simulink model "Steppermotor"  (R2025b)
settings: Solver=FixedStepAuto  StartTime=0.0  StopTime=inf  FixedStep=0.05  RelTol=1e-3  EnableMultiTasking=on
libraries: raspberrypiBasiclib x5, simulink x3, raspberrypiNetworklib x1
settings Model: ExtModeTrigDuration=2  Creator=ioannisgeorgilas  LastModifiedBy=maiaguo
settings SolverCC: PositivePriorityOrder=on
settings OptimizationCC: EnhancedBackFolding=on  PassReuseOutputArgsAs=Individual arguments  ZeroExternalMemoryAtStartup=off  ZeroInternalMemoryAtStartup=off  MaxStackSize=200000  OptimizeBlockOrder=speed  DifferentSizesBufferReuse=on  OptimizationCustomize=off  EfficientTunableParamExpr=on
settings DebuggingCC: ParameterTunabilityLossMsg=error
settings HardwareCC: ProdBitPerPointer=32.0  ProdBitPerSizeT=32.0  ProdBitPerPtrDiffT=32.0  ProdLargestAtomicInteger=Long  ProdLargestAtomicFloat=Double  ProdWordSize=32.0  ProdLongLongMode=on  ProdHWDeviceType=ARM Compatible->ARM Cortex-A (32-bit)
settings RTWCC: SystemTargetFile=ert.tlc  HardwareBoard=Raspberry Pi  TLCOptions="-aInlineSetEventsForThisBaseRateFcn=TLC_FALSE -aSuppressMultiTaskScheduler=TLC_FALSE  -aRateBasedStepFcn=0"  TemplateMakefile=ert_default_tmf  Toolchain=GNU GCC Embedded Linux  BuildConfiguration=Faster Runs  Description=Embedded Coder
settings CodeAppCC: ForceParamTrailComments=on  IgnoreCustomStorageClasses=off  OperatorAnnotations=on  SimulinkDataObjDesc=on  SFDataObjDesc=on  InsertBlockDesc=on
settings ERTTargetCC: ExtModeTransport=2.0  ExtModeStaticAlloc=on  ExtModeMexFile=ext_xcp  ExtModeIntrfLevel=Level2 - Open  InlinedParameterPlacement=Hierarchical  CodeReplacementLibrary=ARM Cortex-A CMSIS  SupportVariableSizeSignals=on

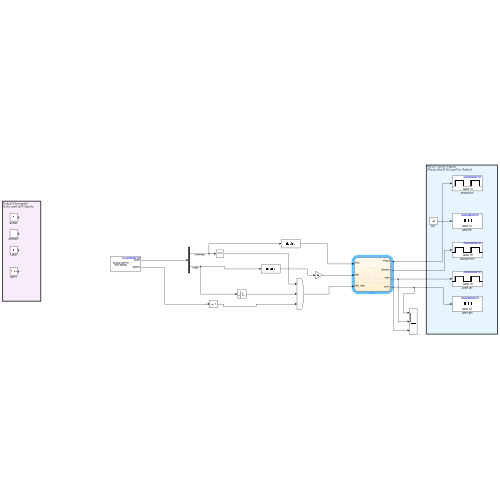
[thumbnail: Simulink's stored preview of the top-level diagram]
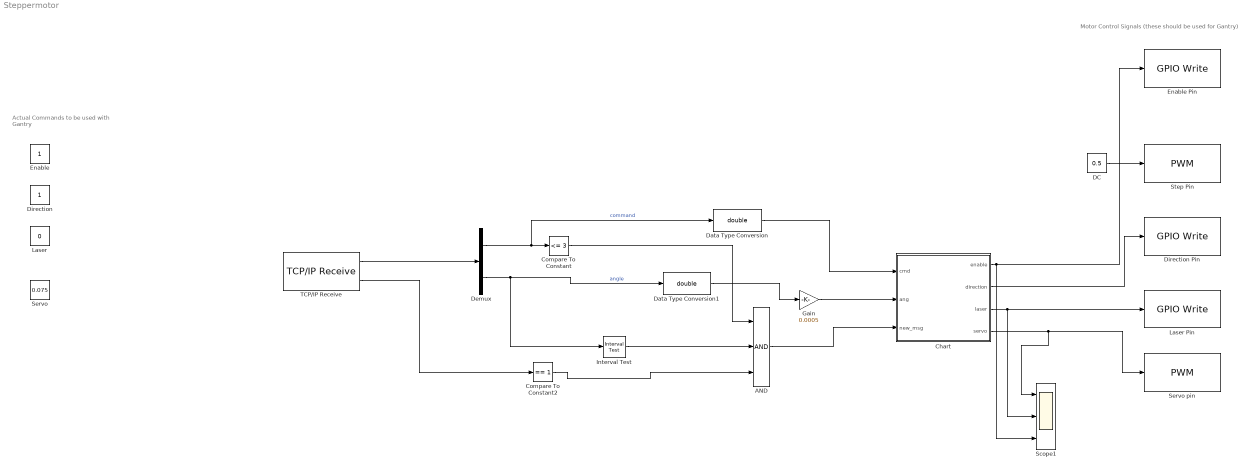
== system Steppermotor ==
  note: Actual Commands
      | to be used with Gantry
  note: Motor Control Signals
      | (these should be used for Gantry)
  AND : Logic  Inputs=3  IconShape=distinctive  AllPortsSameDT=off  OutDataTypeStr=boolean
  Chart : Stateflow chart  TreatAsAtomicUnit=on
  Compare To Constant : simulink/Logic and Bit Operations/Compare To Constant  relop=<=  const=3  OutDataTypeStr=boolean
  Compare To Constant2 : simulink/Logic and Bit Operations/Compare To Constant  relop===  const=1  OutDataTypeStr=boolean
  DC : Constant  Value=0.5  SampleTime=-1
  Data Type Conversion : DataTypeConversion  OutDataTypeStr=double  SaturateOnIntegerOverflow=off  RndMeth=Floor
  Data Type Conversion1 : DataTypeConversion  OutDataTypeStr=double  SaturateOnIntegerOverflow=off  RndMeth=Floor
  Demux : Demux  Outputs=2
  Direction : Constant  SampleTime=-1
  Direction Pin : raspberrypiBasiclib/GPIO Write  BoardProperty=Pi 3 Model B+  gpio=18  blockPlatform=Raspberry Pi  PinNumber=17  board=[]  direction=[]
  Enable : Constant  SampleTime=-1
  Enable Pin : raspberrypiBasiclib/GPIO Write  BoardProperty=Pi 3 Model B+  gpio=14  blockPlatform=Raspberry Pi  PinNumber=17  board=[]  direction=[]
  Gain : Gain  Gain=0.0005
  Interval Test : simulink/Logic and Bit Operations/Interval Test  IntervalClosedRight=on  uplimit=200  IntervalClosedLeft=on  lowlimit=100  OutDataTypeStr=boolean
  Laser : Constant  Value=0  SampleTime=-1
  Laser Pin : raspberrypiBasiclib/GPIO Write  BoardProperty=Pi 3 Model B+  gpio=16  blockPlatform=Raspberry Pi  PinNumber=17  board=[]  direction=[]
  Scope1 : Scope  NumInputPorts=3
      settings: ActiveDisplayYMinimum=-10.948026412434768  ActiveDisplayYMaximum=10.835865541104447
  Servo : Constant  Value=0.075  SampleTime=-1
  Servo pin : raspberrypiBasiclib/PWM  board=Pi 3 Model B+  Pin_=12  Frequency=50  blockPlatform=Raspberry Pi
  Step Pin : raspberrypiBasiclib/PWM  board=Pi 3 Model B+  Pin_=15  Frequency=160  blockPlatform=Raspberry Pi
  TCP/IP Receive : raspberrypiNetworklib/TCP//IP Receive  Mode_=Server  LocalServerPort_=25000  RemoteAddr_=127.0.0.1  RemoteServerPort_=25000  DataType_=uint8  DataSize_=2  SampleTime_=0.05  SimulateUsing=Code generation  ClientPortBindingSelection_=off  ClientPortToBind_=35000  BlockingMode_=off  BlockTimeout_=0.1  BlockPlatform=RASPBERRYPI
  wires:
  DC/1 -> Step Pin/1
  TCP/IP Receive/1 -> Demux/1
  TCP/IP Receive/2 -> Compare To Constant2/1
  Demux/1 -> Data Type Conversion/1, Compare To Constant/1  "command"
  Compare To Constant/1 -> AND/1
  Demux/2 -> Interval Test/1, Data Type Conversion1/1  "angle"
  Interval Test/1 -> AND/2
  AND/1 -> Chart/3(new_msg)
  Data Type Conversion1/1 -> Gain/1
  Data Type Conversion/1 -> Chart/1(cmd)
  Chart/1(enable) -> Scope1/3, Enable Pin/1
  Chart/2(direction) -> Direction Pin/1
  Chart/3(laser) -> Scope1/2, Laser Pin/1
  Chart/4(servo) -> Scope1/1, Servo pin/1
  Compare To Constant2/1 -> AND/3
  Gain/1 -> Chart/2(ang)

== stateflow chart Steppermotor/Chart ==
  state connected
    en: silent = 0;
    du: silent = silent +1;
    state forward
      en: enable = 0;
      direction = 1;
      laser = 0;
      servo = 0.075;
    state stopped
      en: enable = 1;
      laser = 0;
      servo = 0.075;
    state backward
      en: enable = 0;
      direction = 0;
      laser = 0;
      servo = 0.075;
    state firing
      en: enable = 1;
      laser = 1;
      servo = ang;
    connected -> (junction 29) [order 1] : [new_msg==1]{silent=0;}
    (junction 29) -> firing [order 4] : [cmd==2]
    (junction 29) -> stopped [order 1] : [cmd==3]
    (junction 29) -> backward [order 3] : [cmd==1]
    (junction 29) -> forward [order 2] : [cmd==0]
    (default) -> forward
  state lost_link
    en: enable = 1;
    laser = 0;
    servo = 0.075;
  (default) -> connected
  connected -> lost_link [order 1] : [silent>10]
  lost_link -> connected : [new_msg==1]
  data: cmd input; ang input; new_msg input; enable output =1; direction output =0; laser output =0; servo output =0.075; silent local =0
